simulink library "test_sequence_lib"  (R2018b)
settings: Solver=VariableStepAuto  StartTime=0.0  StopTime=10.0  RelTol=1e-3
undefined symbols (not defined in the file): C_BBU, C_DC, C_LV_BASE, C_MV_BASE, C_MV_CELL, F_NOM, ILV_MAX, ILV_MIN, IMV_MAX, IMV_MIN, INVERTER_COUNT, L_HV_BASE, L_LV_BASE, L_MV_BASE, N_CELLS_PER_STRING, N_DCDC_XFMR, N_GSU, N_MVT, plecs, r_BBU, V_LVDC_NOM, VHV_NOM, Z_HV_BASE
libraries: simulink x53, $bdroot x2
settings Model: Creator=HussamAlatrash  LastModifiedBy=ahhei
settings DataIOCC: ReturnWorkspaceOutputs=on
settings DebuggingCC: UnconnectedInputMsg=none  UnconnectedOutputMsg=none  UnconnectedLineMsg=none
settings ModelReferenceCC: EnableRefExpFcnMdlSchedulingChecks=off
settings RTWCC: Description=Generic Real-Time Target
settings ConfigComp: CovBoundaryAbsTol=1.0e-5

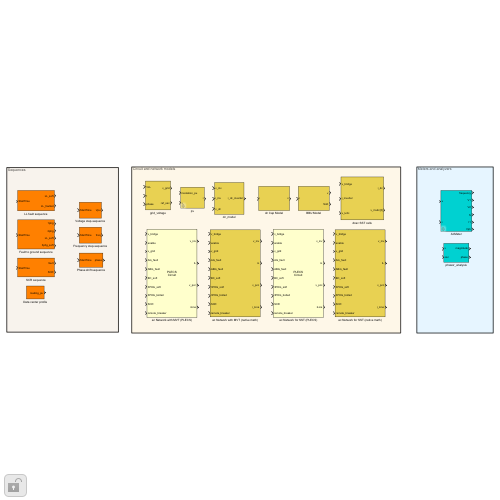
[thumbnail: Simulink's stored preview of the top-level diagram]
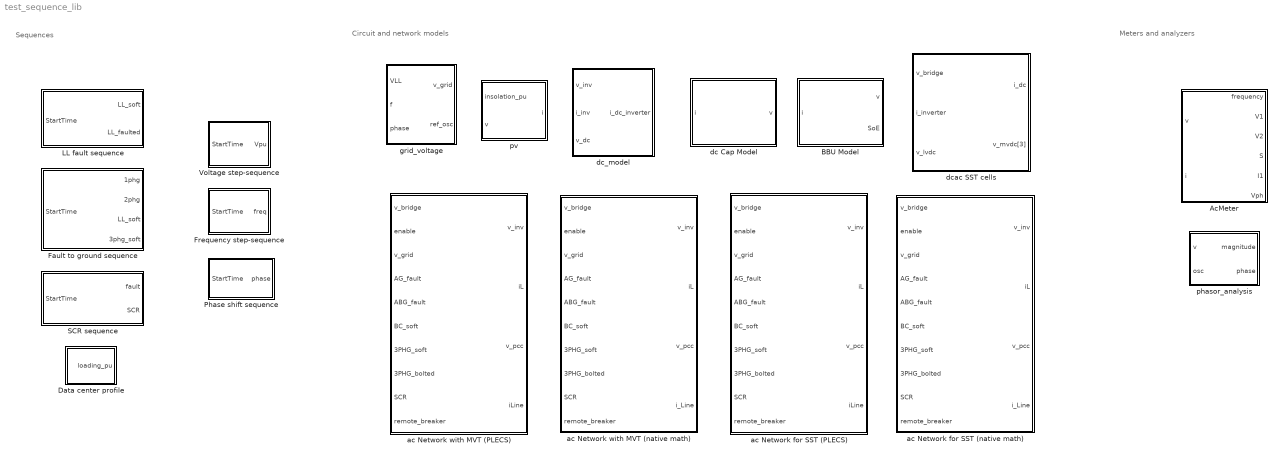
== system test_sequence_lib ==
  note: Meters and analyzers
  note: Circuit and network models
  note: Sequences
  AcMeter : Subsystem  mask{VllRated=VHV_NOM}
      mask prompts: VllRated "Rated line voltage"
  BBU Model : Subsystem
  Data center profile : Subsystem
  Fault to ground sequence : Subsystem
  Frequency step-sequence : Subsystem
  LL fault sequence : Subsystem
  Phase shift sequence : Subsystem
  SCR sequence : Subsystem
  Voltage step-sequence : Subsystem
  ac Network for SST (PLECS) : Subsystem  LoadFcn=plecs('sl', 200);  InitFcn=plecs('sl', 214);  StartFcn=plecs('sl', 208);  StopFcn=plecs('sl', 209);  mask(PlecsCircuit){PLECSData=<binary blob, 8356 chars, not shown>}
      mask prompts: PLECSData "PLECS Data (Do not delete or modify!)"
      mask init:
      | % PLACE CUSTOM INITIALIZATIONS ABOVE
      | % DO NOT REMOVE
      | plecs('sl', 215);
      | % DO NOT REMOVE
      settings: CopyFcn=plecs('sl', 203);  DeleteFcn=plecs('sl', 205);  UndoDeleteFcn=plecs('sl', 206);  PreSaveFcn=plecs('sl', 211);  PostSaveFcn=plecs('sl', 201);  NameChangeFcn=plecs('sl', 210);  DestroyFcn=plecs('sl', 207);  PreCopyFcn=plecs('sl', 216);  OpenFcn=plecs('sl', 202);  ErrorFcn=plerrorfcn
      mask Help: eval('plecs(''help'', ''qthelp:///creatingacircuit.html'')')
      mask Display: disp('PLECS\nCircuit')
  ac Network for SST (native math) : Subsystem
  ac Network with MVT (PLECS) : Subsystem  LoadFcn=plecs('sl', 200);  InitFcn=plecs('sl', 214);  StartFcn=plecs('sl', 208);  StopFcn=plecs('sl', 209);  mask(PlecsCircuit){PLECSData=<binary blob, 8620 chars, not shown>}
      mask prompts: PLECSData "PLECS Data (Do not delete or modify!)"
      mask init:
      | % PLACE CUSTOM INITIALIZATIONS ABOVE
      | % DO NOT REMOVE
      | plecs('sl', 215);
      | % DO NOT REMOVE
      settings: CopyFcn=plecs('sl', 203);  DeleteFcn=plecs('sl', 205);  UndoDeleteFcn=plecs('sl', 206);  PreSaveFcn=plecs('sl', 211);  PostSaveFcn=plecs('sl', 201);  NameChangeFcn=plecs('sl', 210);  DestroyFcn=plecs('sl', 207);  PreCopyFcn=plecs('sl', 216);  OpenFcn=plecs('sl', 202);  ErrorFcn=plerrorfcn
      mask Help: eval('plecs(''help'', ''qthelp:///creatingacircuit.html'')')
      mask Display: disp('PLECS\nCircuit')
  ac Network with MVT (native math) : Subsystem
  dc Cap Model : Subsystem
  dc_model : Subsystem
  dcac SST cells : Subsystem
  grid_voltage : Subsystem
  phasor_analysis : Subsystem
  pv : Subsystem  mask{VopenCircuit=1500, IshortCircuit=1000}
      mask prompts: VopenCircuit "Open Circuit Voltage"; IshortCircuit "Short Circuit Current"

== system test_sequence_lib/AcMeter ==
  v : Inport
  i : Inport  Port=2
  Conj : Math  Operator=conj  SaturateOnIntegerOverflow=on
  PLL_3ph : Subsystem
  Product : Product
  RMS calculator : Subsystem
  Sum of Elements : Sum  Inputs=+
  overVnom : Gain  Gain=1/VllRated
  phasor_analysis : Subsystem
  phasor_analysis1 : $bdroot/AcMeter/phasor_analysis  SystemSampleTime=-1  EmptyChoice=off  PassThrough=off  PassThroughVariantControl=(default)  EmptyChoiceVariantControl=(default)  Latency=0  AutoFrameSizeCalculation=off
  sqrt(3) : Gain  Gain=sqrt(3)
  sqrt(3)1 : Gain  Gain=sqrt(3)
  frequency : Outport
  V1 : Outport  Port=2
  V2 : Outport  Port=3
  S : Outport  Port=4
  I1 : Outport  Port=5
  Vph : Outport  Port=6
  wires:
  sqrt(3)/1 -> V1/1  "Vpve_LL"
  i/1 -> phasor_analysis1/1
  sqrt(3)1/1 -> V2/1  "Vnve_LL"
  phasor_analysis1/2 -> I1/1  "Ipve"
  phasor_analysis/3(nve) -> sqrt(3)1/1
  phasor_analysis/2(pve) -> sqrt(3)/1  "Vpve_LN"
  Product/1 -> Sum of Elements/1
  Conj/1 -> Product/2
  overVnom/1 -> PLL_3ph/1(ref)
  phasor_analysis1/1 -> Conj/1
  PLL_3ph/1(freq) -> frequency/1
  v/1 -> overVnom/1, phasor_analysis/1(in), RMS calculator/1(in[3])
  Sum of Elements/1 -> S/1  "S"
  phasor_analysis/1(perPh) -> Product/1
  PLL_3ph/2(osc[3]) -> phasor_analysis1/2, phasor_analysis/2(osc)
  RMS calculator/1(out[3]) -> Vph/1

== system test_sequence_lib/BBU Model ==
  note: this filter accounts for different caps on the bus
  i : Inport
  Constant : Constant  Value=V_LVDC_NOM
  Constant1 : Constant  Value=0.5
  Gain : Gain  Gain=4/V_LVDC_NOM
  Integrator : Integrator  InitialCondition=V_LVDC_NOM
  Saturation : Saturate  UpperLimit=1.1  LowerLimit=-0.1
  Sum : Sum  Inputs=|++
  Sum1 : Sum  Inputs=|-+
  Sum2 : Sum  Inputs=|++
  Transfer Fcn : TransferFcn  Denominator=[0.1e-3 1]
  over_BBU_capacitance : Gain  Gain=1/C_BBU
  r_BBU : Gain  Gain=r_BBU
  v : Outport
  SoE : Outport  Port=2
  wires:
  over_BBU_capacitance/1 -> Integrator/1
  Integrator/1 -> Sum/1, Sum1/2
  i/1 -> r_BBU/1, over_BBU_capacitance/1
  r_BBU/1 -> Transfer Fcn/1
  Sum/1 -> v/1
  Transfer Fcn/1 -> Sum/2
  Gain/1 -> Sum2/1
  Sum1/1 -> Gain/1
  Constant/1 -> Sum1/1
  Sum2/1 -> Saturation/1
  Constant1/1 -> Sum2/2
  Saturation/1 -> SoE/1

== system test_sequence_lib/Data center profile ==
  Compare To Constant : simulink/Logic and Bit Operations/Compare To Constant  relop=<  const=0.2  OutDataTypeStr=boolean
  Compare To Constant1 : simulink/Logic and Bit Operations/Compare To Constant  relop=<  const=0.8  OutDataTypeStr=boolean
  Compare To Constant2 : simulink/Logic and Bit Operations/Compare To Constant  relop=<  const=0.5  OutDataTypeStr=boolean
  Constant16 : Constant
  Constant17 : Constant  Value=0.1
  Constant18 : Constant  Value=0.1
  Constant19 : Constant  Value=1.5
  Floor : Rounding
  Floor1 : Rounding
  Integrator : Integrator
  Integrator1 : Integrator
  Sum : Sum  Inputs=|+-
  Sum4 : Sum  Inputs=|+-
  Switch : Switch  Criteria=u2 > Threshold
  Switch1 : Switch  Criteria=u2 > Threshold
  Switch2 : Switch  Criteria=u2 > Threshold
  cycle_frequency : Constant  Value=0.5
  pulse_frequency : Constant  Value=10
  loading_pu : Outport
  wires:
  Integrator1/1 -> Floor1/1, Sum4/1
  Floor/1 -> Sum/2
  Integrator/1 -> Sum/1, Floor/1
  Constant16/1 -> Switch/1
  Floor1/1 -> Sum4/2
  Constant17/1 -> Switch1/3  "checkpoint"
  Compare To Constant/1 -> Switch/2
  Constant18/1 -> Switch2/3
  Compare To Constant1/1 -> Switch1/2
  Sum4/1 -> Compare To Constant2/1
  Sum/1 -> Compare To Constant1/1, Compare To Constant/1
  cycle_frequency/1 -> Integrator/1
  pulse_frequency/1 -> Integrator1/1
  Switch1/1 -> Switch/3
  Compare To Constant2/1 -> Switch2/2
  Switch2/1 -> Switch1/1  "training ripple"
  Constant19/1 -> Switch2/1
  Switch/1 -> loading_pu/1

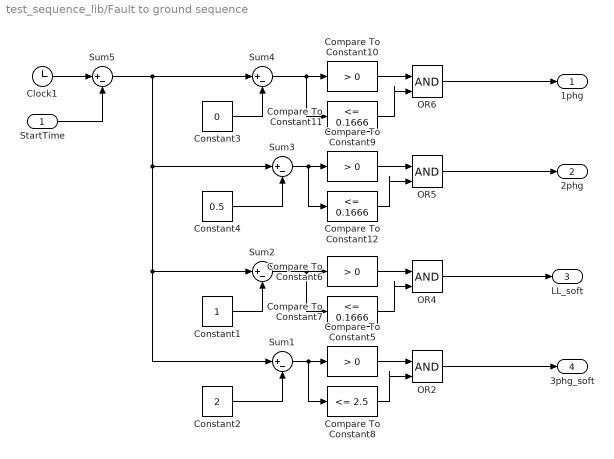
== system test_sequence_lib/Fault to ground sequence ==
  StartTime : Inport
  Clock1 : Clock
  Compare To Constant{5..6,9..10} (4 alike) : simulink/Logic and Bit Operations/Compare To Constant  relop=>  const=0  OutDataTypeStr=boolean
  Compare To Constant11 : simulink/Logic and Bit Operations/Compare To Constant  relop=<=  const=0.1666  OutDataTypeStr=boolean
  Compare To Constant12 : simulink/Logic and Bit Operations/Compare To Constant  relop=<=  const=0.1666  OutDataTypeStr=boolean
  Compare To Constant7 : simulink/Logic and Bit Operations/Compare To Constant  relop=<=  const=0.1666  OutDataTypeStr=boolean
  Compare To Constant8 : simulink/Logic and Bit Operations/Compare To Constant  relop=<=  const=2.5  OutDataTypeStr=boolean
  Constant1 : Constant
  Constant2 : Constant  Value=2
  Constant3 : Constant  Value=0
  Constant4 : Constant  Value=0.5
  OR{2,4..6} (4 alike) : Logic  IconShape=distinctive  AllPortsSameDT=off  OutDataTypeStr=boolean
  Sum{1..5} (5 alike) : Sum  Inputs=|+-
  1phg : Outport
  2phg : Outport  Port=2
  LL_soft : Outport  Port=3
  3phg_soft : Outport  Port=4
  wires:
  Compare To Constant6/1 -> OR4/1
  Compare To Constant8/1 -> OR2/2
  Compare To Constant7/1 -> OR4/2
  Sum2/1 -> Compare To Constant7/1, Compare To Constant6/1
  Sum4/1 -> Compare To Constant10/1, Compare To Constant11/1
  Constant1/1 -> Sum2/2
  Sum1/1 -> Compare To Constant8/1, Compare To Constant5/1
  Compare To Constant5/1 -> OR2/1
  Sum5/1 -> Sum4/1, Sum3/1, Sum2/1, Sum1/1
  Compare To Constant12/1 -> OR5/2
  Sum3/1 -> Compare To Constant9/1, Compare To Constant12/1
  Constant2/1 -> Sum1/2
  Compare To Constant10/1 -> OR6/1
  OR6/1 -> 1phg/1
  Compare To Constant11/1 -> OR6/2
  Compare To Constant9/1 -> OR5/1
  Constant4/1 -> Sum3/2
  Constant3/1 -> Sum4/2
  OR4/1 -> LL_soft/1
  OR5/1 -> 2phg/1
  OR2/1 -> 3phg_soft/1
  Clock1/1 -> Sum5/1
  StartTime/1 -> Sum5/2

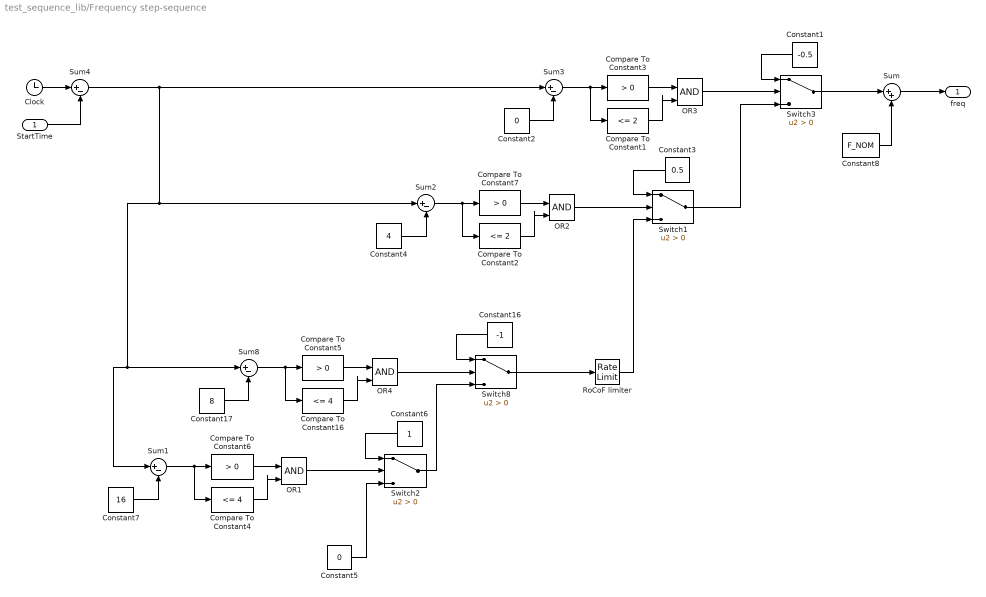
== system test_sequence_lib/Frequency step-sequence ==
  StartTime : Inport
  Clock : Clock
  Compare To Constant1 : simulink/Logic and Bit Operations/Compare To Constant  relop=<=  const=2  OutDataTypeStr=boolean
  Compare To Constant16 : simulink/Logic and Bit Operations/Compare To Constant  relop=<=  const=4  OutDataTypeStr=boolean
  Compare To Constant2 : simulink/Logic and Bit Operations/Compare To Constant  relop=<=  const=2  OutDataTypeStr=boolean
  Compare To Constant{3,5..7} (4 alike) : simulink/Logic and Bit Operations/Compare To Constant  relop=>  const=0  OutDataTypeStr=boolean
  Compare To Constant4 : simulink/Logic and Bit Operations/Compare To Constant  relop=<=  const=4  OutDataTypeStr=boolean
  Constant1 : Constant  Value=-0.5
  Constant16 : Constant  Value=-1
  Constant17 : Constant  Value=8
  Constant2 : Constant  Value=0
  Constant3 : Constant  Value=0.5
  Constant4 : Constant  Value=4
  Constant5 : Constant  Value=0
  Constant6 : Constant
  Constant7 : Constant  Value=16
  Constant8 : Constant  Value=F_NOM
  OR{1..4} (4 alike) : Logic  IconShape=distinctive  AllPortsSameDT=off  OutDataTypeStr=boolean
  RoCoF limiter : RateLimiter  SampleTimeMode=inherited
  Sum : Sum  Inputs=|++
  Sum{1..4,8} (5 alike) : Sum  Inputs=|+-
  Switch{1..3,8} (4 alike) : Switch  Criteria=u2 > Threshold
  freq : Outport
  wires:
  Switch2/1 -> Switch8/3
  Constant16/1 -> Switch8/1
  OR4/1 -> Switch8/2
  Compare To Constant5/1 -> OR4/1
  Sum8/1 -> Compare To Constant5/1, Compare To Constant16/1
  Constant17/1 -> Sum8/2
  Compare To Constant16/1 -> OR4/2
  Constant5/1 -> Switch2/3
  Constant6/1 -> Switch2/1
  OR1/1 -> Switch2/2
  Compare To Constant6/1 -> OR1/1
  Sum1/1 -> Compare To Constant6/1, Compare To Constant4/1
  Constant7/1 -> Sum1/2
  Compare To Constant4/1 -> OR1/2
  Compare To Constant2/1 -> OR2/2
  Constant4/1 -> Sum2/2
  Sum2/1 -> Compare To Constant2/1, Compare To Constant7/1
  Compare To Constant7/1 -> OR2/1
  OR2/1 -> Switch1/2
  Constant3/1 -> Switch1/1
  Switch3/1 -> Sum/1
  Compare To Constant1/1 -> OR3/2
  Constant2/1 -> Sum3/2
  Sum3/1 -> Compare To Constant1/1, Compare To Constant3/1
  Compare To Constant3/1 -> OR3/1
  OR3/1 -> Switch3/2
  Constant1/1 -> Switch3/1
  Sum4/1 -> Sum1/1, Sum8/1, Sum2/1, Sum3/1
  Switch1/1 -> Switch3/3
  Clock/1 -> Sum4/1
  StartTime/1 -> Sum4/2
  Switch8/1 -> RoCoF limiter/1
  RoCoF limiter/1 -> Switch1/3
  Sum/1 -> freq/1
  Constant8/1 -> Sum/2

== system test_sequence_lib/LL fault sequence ==
  StartTime : Inport
  Clock : Clock
  Compare To Constant1 : simulink/Logic and Bit Operations/Compare To Constant  relop=>  const=0  OutDataTypeStr=boolean
  Compare To Constant2 : simulink/Logic and Bit Operations/Compare To Constant  relop=>  const=0  OutDataTypeStr=boolean
  Compare To Constant3 : simulink/Logic and Bit Operations/Compare To Constant  relop=<=  const=0.1666  OutDataTypeStr=boolean
  Compare To Constant4 : simulink/Logic and Bit Operations/Compare To Constant  relop=<=  const=0.1666  OutDataTypeStr=boolean
  Constant11 : Constant  Value=0.5
  OR1 : Logic  IconShape=distinctive  AllPortsSameDT=off  OutDataTypeStr=boolean
  OR3 : Logic  IconShape=distinctive  AllPortsSameDT=off  OutDataTypeStr=boolean
  Sum : Sum  Inputs=|+-
  Sum8 : Sum  Inputs=|+-
  LL_soft : Outport
  LL_faulted : Outport  Port=2
  wires:
  Compare To Constant2/1 -> OR3/1
  Compare To Constant4/1 -> OR1/2
  OR1/1 -> LL_faulted/1
  Compare To Constant3/1 -> OR3/2
  OR3/1 -> LL_soft/1
  Compare To Constant1/1 -> OR1/1
  Clock/1 -> Sum/1
  StartTime/1 -> Sum/2
  Sum8/1 -> Compare To Constant1/1, Compare To Constant4/1
  Sum/1 -> Compare To Constant2/1, Compare To Constant3/1, Sum8/1
  Constant11/1 -> Sum8/2

== system test_sequence_lib/Phase shift sequence ==
  StartTime : Inport
  Clock3 : Clock
  Compare To Constant13 : simulink/Logic and Bit Operations/Compare To Constant  relop=<=  const=1  OutDataTypeStr=boolean
  Compare To Constant14 : simulink/Logic and Bit Operations/Compare To Constant  relop=>  const=0  OutDataTypeStr=boolean
  Constant5 : Constant  Value=-25*pi/180
  Constant7 : Constant  Value=0
  OR7 : Logic  IconShape=distinctive  AllPortsSameDT=off  OutDataTypeStr=boolean
  Sum5 : Sum  Inputs=|+-
  Switch3 : Switch  Criteria=u2 > Threshold
  phase : Outport
  wires:
  OR7/1 -> Switch3/2
  Sum5/1 -> Compare To Constant13/1, Compare To Constant14/1
  Constant7/1 -> Switch3/3
  Constant5/1 -> Switch3/1
  Compare To Constant14/1 -> OR7/1
  Compare To Constant13/1 -> OR7/2
  Switch3/1 -> phase/1
  Clock3/1 -> Sum5/1
  StartTime/1 -> Sum5/2

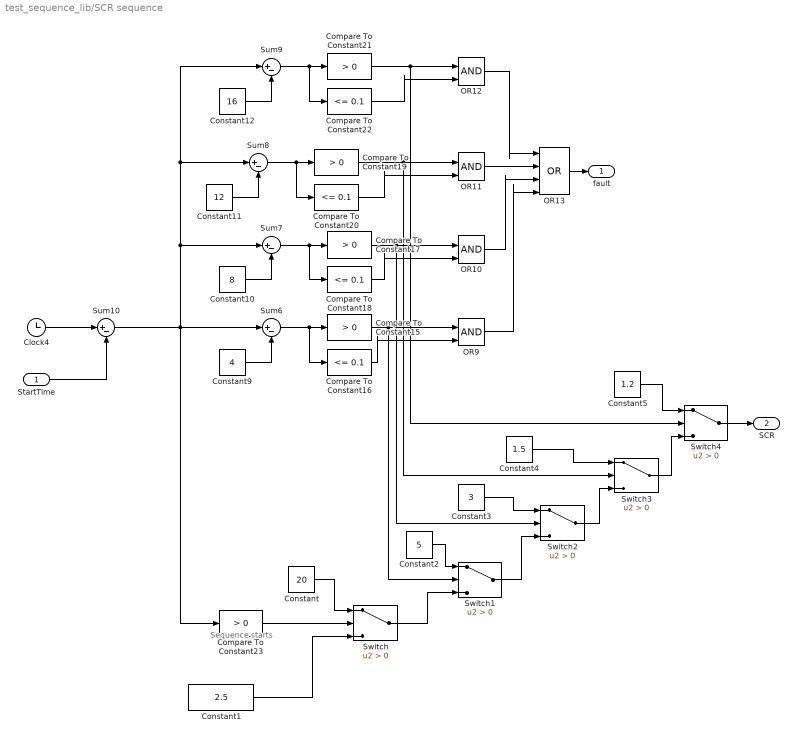
== system test_sequence_lib/SCR sequence ==
  note: Sequence starts
  StartTime : Inport
  Clock4 : Clock
  Compare To Constant{15,17,19,21,23} (5 alike) : simulink/Logic and Bit Operations/Compare To Constant  relop=>  const=0  OutDataTypeStr=boolean
  Compare To Constant{16,18,20,22} (4 alike) : simulink/Logic and Bit Operations/Compare To Constant  relop=<=  const=0.1  OutDataTypeStr=boolean
  Constant : Constant  Value=20
  Constant1 : Constant  Value=2.5
  Constant10 : Constant  Value=8
  Constant11 : Constant  Value=12
  Constant12 : Constant  Value=16
  Constant2 : Constant  Value=5
  Constant3 : Constant  Value=3
  Constant4 : Constant  Value=1.5
  Constant5 : Constant  Value=1.2
  Constant9 : Constant  Value=4
  OR{9..12} (4 alike) : Logic  IconShape=distinctive  AllPortsSameDT=off  OutDataTypeStr=boolean
  OR13 : Logic  Operator=OR  Inputs=4  IconShape=distinctive  AllPortsSameDT=off  OutDataTypeStr=boolean
  Sum{6..10} (5 alike) : Sum  Inputs=|+-
  Switch{,1..4} (5 alike) : Switch  Criteria=u2 > Threshold
  fault : Outport
  SCR : Outport  Port=2
  wires:
  OR13/1 -> fault/1
  Sum10/1 -> Sum9/1, Sum8/1, Sum7/1, Compare To Constant23/1, Sum6/1
  Constant11/1 -> Sum8/2
  Compare To Constant17/1 -> Switch2/2, OR10/1
  Sum9/1 -> Compare To Constant22/1, Compare To Constant21/1
  Clock4/1 -> Sum10/1
  Compare To Constant19/1 -> Switch3/2, OR11/1
  Sum8/1 -> Compare To Constant20/1, Compare To Constant19/1
  StartTime/1 -> Sum10/2
  Compare To Constant21/1 -> OR12/1, Switch4/2
  Compare To Constant15/1 -> Switch1/2, OR9/1
  Sum7/1 -> Compare To Constant18/1, Compare To Constant17/1
  Sum6/1 -> Compare To Constant16/1, Compare To Constant15/1
  Compare To Constant20/1 -> OR11/2
  Constant10/1 -> Sum7/2
  Compare To Constant18/1 -> OR10/2
  Constant12/1 -> Sum9/2
  Compare To Constant22/1 -> OR12/2
  Constant9/1 -> Sum6/2
  Compare To Constant16/1 -> OR9/2
  Compare To Constant23/1 -> Switch/2
  Constant/1 -> Switch/1
  Constant1/1 -> Switch/3
  Switch/1 -> Switch1/3
  OR12/1 -> OR13/1
  OR11/1 -> OR13/2
  OR10/1 -> OR13/3
  OR9/1 -> OR13/4
  Switch1/1 -> Switch2/3
  Switch2/1 -> Switch3/3
  Switch3/1 -> Switch4/3
  Constant2/1 -> Switch1/1
  Constant3/1 -> Switch2/1
  Constant4/1 -> Switch3/1
  Constant5/1 -> Switch4/1
  Switch4/1 -> SCR/1

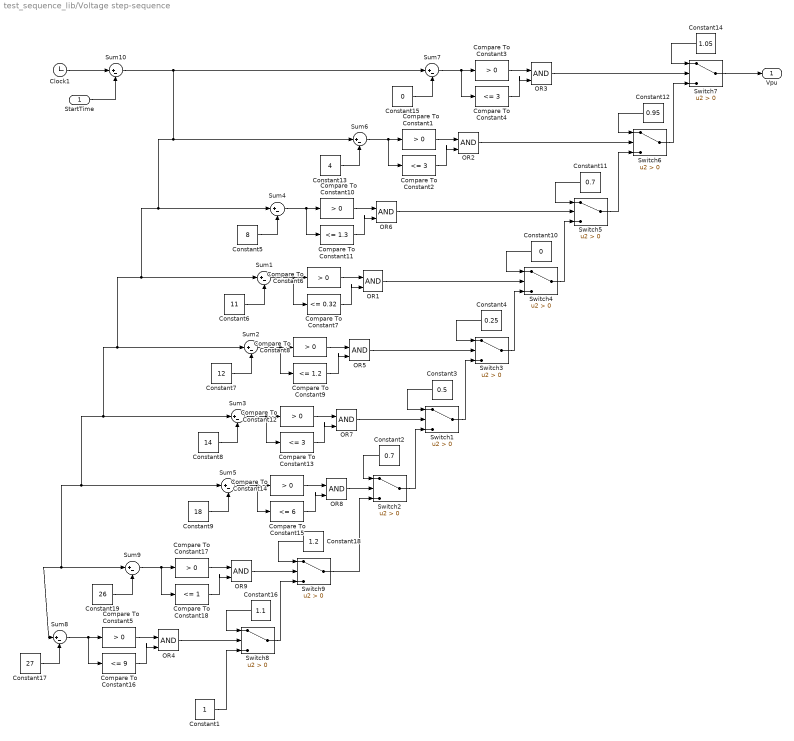
== system test_sequence_lib/Voltage step-sequence ==
  StartTime : Inport
  Clock1 : Clock
  Compare To Constant{1,3,5..6,8,10,12,14,17} (9 alike) : simulink/Logic and Bit Operations/Compare To Constant  relop=>  const=0  OutDataTypeStr=boolean
  Compare To Constant11 : simulink/Logic and Bit Operations/Compare To Constant  relop=<=  const=1.3  OutDataTypeStr=boolean
  Compare To Constant13 : simulink/Logic and Bit Operations/Compare To Constant  relop=<=  const=3  OutDataTypeStr=boolean
  Compare To Constant15 : simulink/Logic and Bit Operations/Compare To Constant  relop=<=  const=6  OutDataTypeStr=boolean
  Compare To Constant16 : simulink/Logic and Bit Operations/Compare To Constant  relop=<=  const=9  OutDataTypeStr=boolean
  Compare To Constant18 : simulink/Logic and Bit Operations/Compare To Constant  relop=<=  const=1  OutDataTypeStr=boolean
  Compare To Constant2 : simulink/Logic and Bit Operations/Compare To Constant  relop=<=  const=3  OutDataTypeStr=boolean
  Compare To Constant4 : simulink/Logic and Bit Operations/Compare To Constant  relop=<=  const=3  OutDataTypeStr=boolean
  Compare To Constant7 : simulink/Logic and Bit Operations/Compare To Constant  relop=<=  const=0.32  OutDataTypeStr=boolean
  Compare To Constant9 : simulink/Logic and Bit Operations/Compare To Constant  relop=<=  const=1.2  OutDataTypeStr=boolean
  Constant1 : Constant
  Constant10 : Constant  Value=0
  Constant11 : Constant  Value=0.7
  Constant12 : Constant  Value=0.95
  Constant13 : Constant  Value=4
  Constant14 : Constant  Value=1.05
  Constant15 : Constant  Value=0
  Constant16 : Constant  Value=1.1
  Constant17 : Constant  Value=27
  Constant18 : Constant  Value=1.2
  Constant19 : Constant  Value=26
  Constant2 : Constant  Value=0.7
  Constant3 : Constant  Value=0.5
  Constant4 : Constant  Value=0.25
  Constant5 : Constant  Value=8
  Constant6 : Constant  Value=11
  Constant7 : Constant  Value=12
  Constant8 : Constant  Value=14
  Constant9 : Constant  Value=18
  OR{1..9} (9 alike) : Logic  IconShape=distinctive  AllPortsSameDT=off  OutDataTypeStr=boolean
  Sum{1..10} (10 alike) : Sum  Inputs=|+-
  Switch{1..9} (9 alike) : Switch  Criteria=u2 > Threshold
  Vpu : Outport
  wires:
  Constant2/1 -> Switch2/1
  Switch2/1 -> Switch1/3
  Switch9/1 -> Switch2/3
  OR7/1 -> Switch1/2
  Constant3/1 -> Switch1/1
  OR8/1 -> Switch2/2
  Sum4/1 -> Compare To Constant10/1, Compare To Constant11/1
  Constant5/1 -> Sum4/2
  OR6/1 -> Switch5/2
  Compare To Constant10/1 -> OR6/1
  Compare To Constant11/1 -> OR6/2
  Compare To Constant7/1 -> OR1/2
  Compare To Constant6/1 -> OR1/1
  Constant6/1 -> Sum1/2
  Sum1/1 -> Compare To Constant7/1, Compare To Constant6/1
  Sum2/1 -> Compare To Constant8/1, Compare To Constant9/1
  Constant7/1 -> Sum2/2
  Compare To Constant8/1 -> OR5/1
  Compare To Constant9/1 -> OR5/2
  Compare To Constant13/1 -> OR7/2
  Compare To Constant12/1 -> OR7/1
  Constant8/1 -> Sum3/2
  Sum3/1 -> Compare To Constant13/1, Compare To Constant12/1
  Sum5/1 -> Compare To Constant14/1, Compare To Constant15/1
  Constant9/1 -> Sum5/2
  Compare To Constant14/1 -> OR8/1
  Compare To Constant15/1 -> OR8/2
  Constant4/1 -> Switch3/1
  OR5/1 -> Switch3/2
  OR1/1 -> Switch4/2
  Constant10/1 -> Switch4/1
  Constant11/1 -> Switch5/1
  Switch1/1 -> Switch3/3
  Switch3/1 -> Switch4/3
  Switch4/1 -> Switch5/3
  Switch5/1 -> Switch6/3
  Constant12/1 -> Switch6/1
  Compare To Constant2/1 -> OR2/2
  Compare To Constant1/1 -> OR2/1
  OR2/1 -> Switch6/2
  Constant13/1 -> Sum6/2
  Sum6/1 -> Compare To Constant2/1, Compare To Constant1/1
  Sum7/1 -> Compare To Constant3/1, Compare To Constant4/1
  Constant15/1 -> Sum7/2
  OR3/1 -> Switch7/2
  Compare To Constant3/1 -> OR3/1
  Compare To Constant4/1 -> OR3/2
  Constant14/1 -> Switch7/1
  Switch6/1 -> Switch7/3
  Switch7/1 -> Vpu/1
  Switch8/1 -> Switch9/3
  Constant18/1 -> Switch9/1
  Sum10/1 -> Sum4/1, Sum1/1, Sum2/1, Sum3/1, Sum5/1, Sum8/1, Sum9/1, Sum6/1, Sum7/1
  Compare To Constant18/1 -> OR9/2
  Compare To Constant17/1 -> OR9/1
  OR9/1 -> Switch9/2
  Constant19/1 -> Sum9/2
  Sum9/1 -> Compare To Constant18/1, Compare To Constant17/1
  Sum8/1 -> Compare To Constant5/1, Compare To Constant16/1
  Constant17/1 -> Sum8/2
  OR4/1 -> Switch8/2
  Compare To Constant5/1 -> OR4/1
  Compare To Constant16/1 -> OR4/2
  Constant16/1 -> Switch8/1
  Constant1/1 -> Switch8/3
  Clock1/1 -> Sum10/1
  StartTime/1 -> Sum10/2

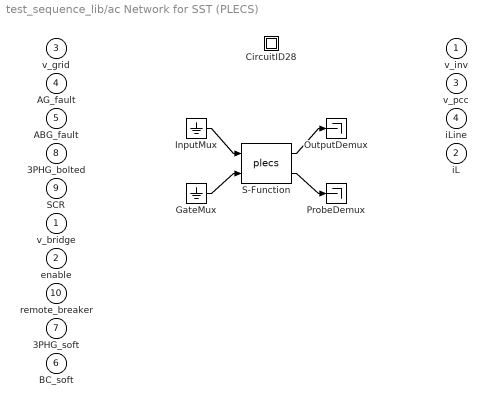
== system test_sequence_lib/ac Network for SST (PLECS) ==
  v_bridge : Inport  PortDimensions=3
  enable : Inport  Port=2  PortDimensions=1
  v_grid : Inport  Port=3  PortDimensions=3
  AG_fault : Inport  Port=4  PortDimensions=1
  ABG_fault : Inport  Port=5  PortDimensions=1
  BC_soft : Inport  Port=6  PortDimensions=1
  3PHG_soft : Inport  Port=7  PortDimensions=1
  3PHG_bolted : Inport  Port=8  PortDimensions=1
  SCR : Inport  Port=9  PortDimensions=1
  remote_breaker : Inport  Port=10  PortDimensions=1
  " CircuitID28 " : Subsystem
  " GateMux " : Ground
  " InputMux " : Ground
  " OutputDemux " : Terminator
  " ProbeDemux " : Terminator
  " S-Function " : S-Function  FunctionName=plecs  SFunctionDeploymentMode=off  EnableBusSupport=off
  v_inv : Outport  PortDimensions=3
  iL : Outport  Port=2  PortDimensions=3
  v_pcc : Outport  Port=3  PortDimensions=3
  iLine : Outport  Port=4  PortDimensions=3
  wires:
  " InputMux "/1 -> " S-Function "/1
  " GateMux "/1 -> " S-Function "/2
  " S-Function "/1 -> " OutputDemux "/1
  " S-Function "/2 -> " ProbeDemux "/1

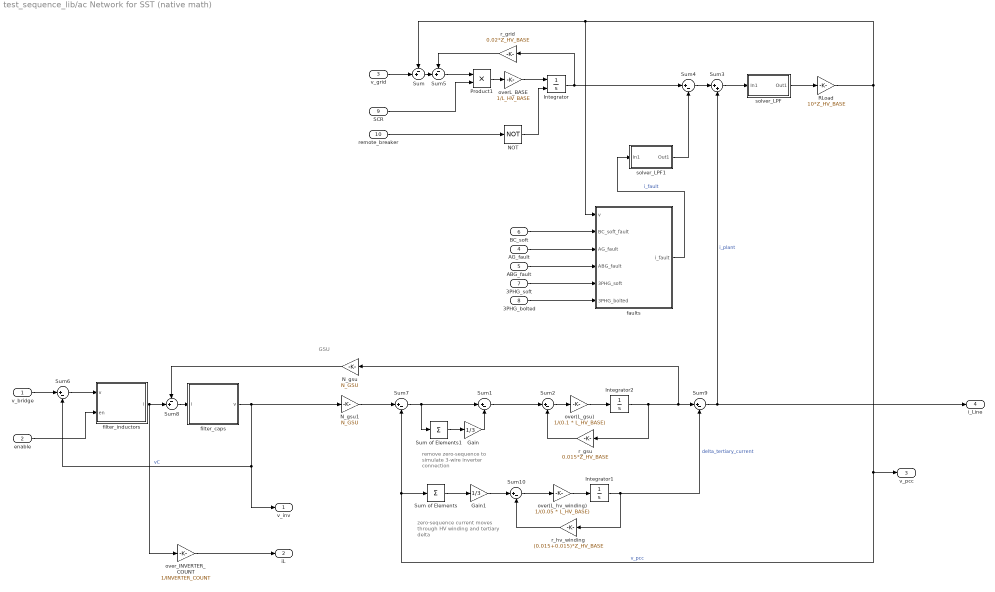
== system test_sequence_lib/ac Network for SST (native math) ==
  note: GSU
  note: remove zero-sequence to simulate 3-wire inverter connection
  note: zero-sequence current moves through HV winding and tertiary delta
  v_bridge : Inport
  enable : Inport  Port=2
  v_grid : Inport  Port=3
  AG_fault : Inport  Port=4
  ABG_fault : Inport  Port=5
  BC_soft : Inport  Port=6
  3PHG_soft : Inport  Port=7
  3PHG_bolted : Inport  Port=8
  SCR : Inport  Port=9
  remote_breaker : Inport  Port=10
  Gain : Gain  Gain=1/3
  Gain1 : Gain  Gain=1/3
  Integrator : Integrator  ExternalReset=level
  Integrator1 : Integrator
  Integrator2 : Integrator
  NOT : Logic  Operator=NOT  IconShape=distinctive  AllPortsSameDT=off  OutDataTypeStr=boolean
  N_gsu : Gain  Gain=N_GSU
  N_gsu1 : Gain  Gain=N_GSU
  Product1 : Product
  RLoad : Gain  Gain=10*Z_HV_BASE
  Sum : Sum  Inputs=-+|
  Sum of Elements : Sum  Inputs=+
  Sum of Elements1 : Sum  Inputs=+
  Sum{1..2,4,6..7,9..10} (7 alike) : Sum  Inputs=|+-
  Sum3 : Sum  Inputs=|++
  Sum5 : Sum  Inputs=-+|
  Sum8 : Sum  Inputs=-+|
  faults : Subsystem
  filter_caps : Subsystem
  filter_inductors : Subsystem
  over(L_gsu) : Gain  Gain=1/(0.1 * L_HV_BASE)
  over(L_hv_winding) : Gain  Gain=1/(0.05 * L_HV_BASE)
  overL_BASE : Gain  Gain=1/L_HV_BASE
  over_INVERTER_COUNT : Gain  Gain=1/INVERTER_COUNT
  r_grid : Gain  Gain=0.02*Z_HV_BASE
  r_gsu : Gain  Gain=0.015*Z_HV_BASE
  r_hv_winding : Gain  Gain=(0.015+0.015)*Z_HV_BASE
  solver_LPF : Subsystem
  solver_LPF1 : Subsystem
  v_inv : Outport
  iL : Outport  Port=2
  v_pcc : Outport  Port=3
  i_Line : Outport  Port=4
  wires:
  3PHG_soft/1 -> faults/5(3PHG_soft)
  Integrator2/1 -> r_gsu/1, N_gsu/1, Sum9/1
  Sum/1 -> Sum5/2
  Sum5/1 -> Product1/1
  v_grid/1 -> Sum/2
  Sum4/1 -> Sum3/1
  NOT/1 -> Integrator/2
  Sum3/1 -> solver_LPF/1(In1)
  r_grid/1 -> Sum5/1
  SCR/1 -> Product1/2
  Product1/1 -> overL_BASE/1
  v_bridge/1 -> Sum6/1
  3PHG_bolted/1 -> faults/6(3PHG_bolted)
  faults/1(i_fault) -> solver_LPF1/1(In1)  "i_fault"
  RLoad/1 -> Sum7/2, Sum of Elements/1, v_pcc/1, Sum/1, faults/1(v)  "v_pcc"
  solver_LPF1/1(Out1) -> Sum4/2
  Integrator/1 -> r_grid/1, Sum4/1
  overL_BASE/1 -> Integrator/1
  remote_breaker/1 -> NOT/1
  solver_LPF/1(Out1) -> RLoad/1
  over(L_gsu)/1 -> Integrator2/1
  Sum7/1 -> Sum of Elements1/1, Sum1/1
  Sum2/1 -> over(L_gsu)/1
  Sum of Elements1/1 -> Gain/1
  Gain/1 -> Sum1/2
  Sum1/1 -> Sum2/1
  r_gsu/1 -> Sum2/2
  Sum6/1 -> filter_inductors/1(v)
  enable/1 -> filter_inductors/2(en)
  filter_inductors/1(i) -> Sum8/2, over_INVERTER_COUNT/1
  Sum8/1 -> filter_caps/1(i)
  filter_caps/1(v) -> v_inv/1, Sum6/2, N_gsu1/1  "vC"
  over_INVERTER_COUNT/1 -> iL/1
  N_gsu1/1 -> Sum7/1
  N_gsu/1 -> Sum8/1
  Sum9/1 -> Sum3/2, i_Line/1  "i_plant"
  over(L_hv_winding)/1 -> Integrator1/1
  Integrator1/1 -> Sum9/2, r_hv_winding/1  "delta_tertiary_current"
  r_hv_winding/1 -> Sum10/2
  Sum10/1 -> over(L_hv_winding)/1
  Sum of Elements/1 -> Gain1/1
  Gain1/1 -> Sum10/1
  BC_soft/1 -> faults/2(BC_soft_fault)
  ABG_fault/1 -> faults/4(ABG_fault)
  AG_fault/1 -> faults/3(AG_fault)

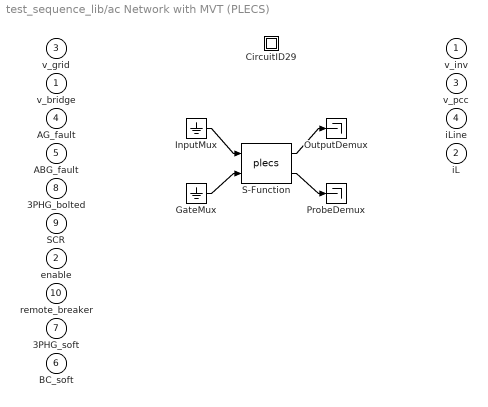
== system test_sequence_lib/ac Network with MVT (PLECS) ==
  v_bridge : Inport  PortDimensions=3
  enable : Inport  Port=2  PortDimensions=1
  v_grid : Inport  Port=3  PortDimensions=3
  AG_fault : Inport  Port=4  PortDimensions=1
  ABG_fault : Inport  Port=5  PortDimensions=1
  BC_soft : Inport  Port=6  PortDimensions=1
  3PHG_soft : Inport  Port=7  PortDimensions=1
  3PHG_bolted : Inport  Port=8  PortDimensions=1
  SCR : Inport  Port=9  PortDimensions=1
  remote_breaker : Inport  Port=10  PortDimensions=1
  " CircuitID29 " : Subsystem
  " GateMux " : Ground
  " InputMux " : Ground
  " OutputDemux " : Terminator
  " ProbeDemux " : Terminator
  " S-Function " : S-Function  FunctionName=plecs  SFunctionDeploymentMode=off  EnableBusSupport=off
  v_inv : Outport  PortDimensions=3
  iL : Outport  Port=2  PortDimensions=3
  v_pcc : Outport  Port=3  PortDimensions=3
  iLine : Outport  Port=4  PortDimensions=3
  wires:
  " InputMux "/1 -> " S-Function "/1
  " GateMux "/1 -> " S-Function "/2
  " S-Function "/1 -> " OutputDemux "/1
  " S-Function "/2 -> " ProbeDemux "/1

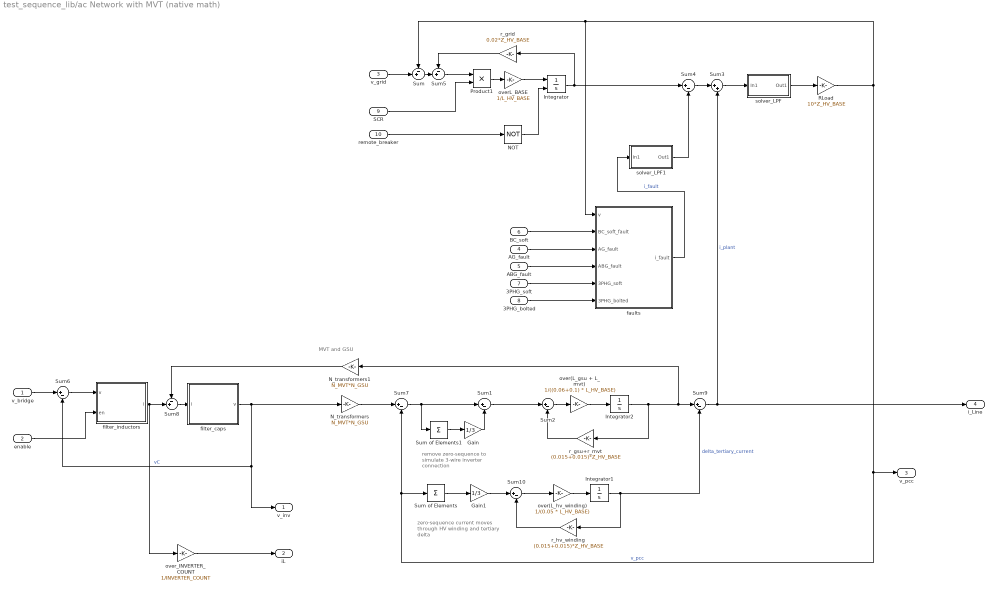
== system test_sequence_lib/ac Network with MVT (native math) ==
  note: MVT and GSU
  note: remove zero-sequence to simulate 3-wire inverter connection
  note: zero-sequence current moves through HV winding and tertiary delta
  v_bridge : Inport
  enable : Inport  Port=2
  v_grid : Inport  Port=3
  AG_fault : Inport  Port=4
  ABG_fault : Inport  Port=5
  BC_soft : Inport  Port=6
  3PHG_soft : Inport  Port=7
  3PHG_bolted : Inport  Port=8
  SCR : Inport  Port=9
  remote_breaker : Inport  Port=10
  Gain : Gain  Gain=1/3
  Gain1 : Gain  Gain=1/3
  Integrator : Integrator  ExternalReset=level
  Integrator1 : Integrator
  Integrator2 : Integrator
  NOT : Logic  Operator=NOT  IconShape=distinctive  AllPortsSameDT=off  OutDataTypeStr=boolean
  N_transformers : Gain  Gain=N_MVT*N_GSU
  N_transformers1 : Gain  Gain=N_MVT*N_GSU
  Product1 : Product
  RLoad : Gain  Gain=10*Z_HV_BASE
  Sum : Sum  Inputs=-+|
  Sum of Elements : Sum  Inputs=+
  Sum of Elements1 : Sum  Inputs=+
  Sum{1..2,4,6..7,9..10} (7 alike) : Sum  Inputs=|+-
  Sum3 : Sum  Inputs=|++
  Sum5 : Sum  Inputs=-+|
  Sum8 : Sum  Inputs=-+|
  faults : Subsystem
  filter_caps : Subsystem
  filter_inductors : Subsystem
  over(L_gsu + L_mvt) : Gain  Gain=1/((0.06+0.1) * L_HV_BASE)
  over(L_hv_winding) : Gain  Gain=1/(0.05 * L_HV_BASE)
  overL_BASE : Gain  Gain=1/L_HV_BASE
  over_INVERTER_COUNT : Gain  Gain=1/INVERTER_COUNT
  r_grid : Gain  Gain=0.02*Z_HV_BASE
  r_gsu+r_mvt : Gain  Gain=(0.015+0.015)*Z_HV_BASE
  r_hv_winding : Gain  Gain=(0.015+0.015)*Z_HV_BASE
  solver_LPF : Subsystem
  solver_LPF1 : Subsystem
  v_inv : Outport
  iL : Outport  Port=2
  v_pcc : Outport  Port=3
  i_Line : Outport  Port=4
  wires:
  3PHG_soft/1 -> faults/5(3PHG_soft)
  Integrator2/1 -> r_gsu+r_mvt/1, N_transformers1/1, Sum9/1
  Sum/1 -> Sum5/2
  Sum5/1 -> Product1/1
  v_grid/1 -> Sum/2
  Sum4/1 -> Sum3/1
  NOT/1 -> Integrator/2
  Sum3/1 -> solver_LPF/1(In1)
  r_grid/1 -> Sum5/1
  SCR/1 -> Product1/2
  Product1/1 -> overL_BASE/1
  v_bridge/1 -> Sum6/1
  3PHG_bolted/1 -> faults/6(3PHG_bolted)
  faults/1(i_fault) -> solver_LPF1/1(In1)  "i_fault"
  RLoad/1 -> Sum7/2, Sum of Elements/1, v_pcc/1, Sum/1, faults/1(v)  "v_pcc"
  solver_LPF1/1(Out1) -> Sum4/2
  Integrator/1 -> r_grid/1, Sum4/1
  overL_BASE/1 -> Integrator/1
  remote_breaker/1 -> NOT/1
  solver_LPF/1(Out1) -> RLoad/1
  over(L_gsu + L_mvt)/1 -> Integrator2/1
  Sum7/1 -> Sum of Elements1/1, Sum1/1
  Sum2/1 -> over(L_gsu + L_mvt)/1
  Sum of Elements1/1 -> Gain/1
  Gain/1 -> Sum1/2
  Sum1/1 -> Sum2/1
  r_gsu+r_mvt/1 -> Sum2/2
  Sum6/1 -> filter_inductors/1(v)
  enable/1 -> filter_inductors/2(en)
  filter_inductors/1(i) -> Sum8/2, over_INVERTER_COUNT/1
  Sum8/1 -> filter_caps/1(i)
  filter_caps/1(v) -> v_inv/1, Sum6/2, N_transformers/1  "vC"
  over_INVERTER_COUNT/1 -> iL/1
  N_transformers/1 -> Sum7/1
  N_transformers1/1 -> Sum8/1
  Sum9/1 -> Sum3/2, i_Line/1  "i_plant"
  over(L_hv_winding)/1 -> Integrator1/1
  Integrator1/1 -> Sum9/2, r_hv_winding/1  "delta_tertiary_current"
  r_hv_winding/1 -> Sum10/2
  Sum10/1 -> over(L_hv_winding)/1
  Sum of Elements/1 -> Gain1/1
  Gain1/1 -> Sum10/1
  BC_soft/1 -> faults/2(BC_soft_fault)
  ABG_fault/1 -> faults/4(ABG_fault)
  AG_fault/1 -> faults/3(AG_fault)

== system test_sequence_lib/dc Cap Model ==
  i : Inport
  Integrator : Integrator  InitialCondition=V_LVDC_NOM
  over_capacitance : Gain  Gain=1/C_DC
  v : Outport
  wires:
  over_capacitance/1 -> Integrator/1
  i/1 -> over_capacitance/1
  Integrator/1 -> v/1

== system test_sequence_lib/dc_model ==
  v_inv : Inport
  i_inv : Inport  Port=2
  v_dc : Inport  Port=3
  Product : Product
  Product1 : Product  Inputs=*/
  Saturation : Saturate  UpperLimit=inf  LowerLimit=10
  Sum of Elements : Sum  Inputs=+
  i_dc_inverter : Outport
  wires:
  v_dc/1 -> Saturation/1
  Sum of Elements/1 -> Product1/1  "P_ac"
  i_inv/1 -> Product/2
  Product/1 -> Sum of Elements/1
  Product1/1 -> i_dc_inverter/1  "i_dc_inverter"
  v_inv/1 -> Product/1
  Saturation/1 -> Product1/2

== system test_sequence_lib/dcac SST cells ==
  note: The three aggregate dc-bus voltages for the three phases do not naturally balance and need this algorithm to do so
  v_bridge : Inport
  i_inverter : Inport  Port=2
  v_lvdc : Inport  Port=3
  Gain1 : Gain  Gain=1/3
  N_cells : Gain  Gain=N_CELLS_PER_STRING
  N_cells1 : Gain  Gain=N_CELLS_PER_STRING
  SST Cell Model : Subsystem
  Sum of Elements : Sum  Inputs=+
  Sum of Elements1 : Sum  Inputs=+
  Sum4 : Sum  Inputs=-+|
  dcdcController : Subsystem
  kRebalance : Gain  Gain=5
  over_N_cells : Gain  Gain=1/N_CELLS_PER_STRING
  i_dc : Outport
  v_mvdc[3] : Outport  Port=2
  wires:
  kRebalance/1 -> dcdcController/3(P_dcdc_ffwd)  "p_string_rebalance"
  N_cells1/1 -> Sum of Elements/1
  N_cells/1 -> v_mvdc[3]/1, Sum4/1, Sum of Elements1/1  "v_mvdc_bus"
  Sum4/1 -> kRebalance/1
  SST Cell Model/2(i_LV) -> N_cells1/1
  Sum of Elements1/1 -> Gain1/1
  dcdcController/1(i_MV_ref) -> SST Cell Model/2(i_MV)
  Gain1/1 -> Sum4/2
  SST Cell Model/1(v_MV_cell) -> N_cells/1, dcdcController/2(v_MV_cell)  "v_mvdc_cell"
  over_N_cells/1 -> SST Cell Model/3(v_ac)
  v_lvdc/1 -> SST Cell Model/1(v_LV), dcdcController/1(v_LV)
  v_bridge/1 -> over_N_cells/1
  Sum of Elements/1 -> i_dc/1  "I_dc_sst"
  i_inverter/1 -> SST Cell Model/4(i_ac)

== system test_sequence_lib/grid_voltage ==
  VLL : Inport
  f : Inport  Port=2
  phase : Inport  Port=3
  Complex to Real-Imag : ComplexToRealImag
  Gain : Gain  Gain=sqrt(2)
  Gain1 : Gain  Gain=1/sqrt(3)
  Product : Product
  oscillator_3ph : Subsystem
  v_grid : Outport
  ref_osc : Outport  Port=2
  wires:
  Complex to Real-Imag/1 -> Gain/1
  oscillator_3ph/1(osc[3]) -> ref_osc/1, Complex to Real-Imag/1
  f/1 -> oscillator_3ph/1(f)
  Gain/1 -> Product/1
  Product/1 -> Gain1/1
  Gain1/1 -> v_grid/1
  VLL/1 -> Product/2
  phase/1 -> oscillator_3ph/2(phase)

== system test_sequence_lib/phasor_analysis ==
  v : Inport
  osc : Inport  Port=2
  Complex to Magnitude-Angle : ComplexToMagnitudeAngle
  Complex to Real-Imag : ComplexToRealImag
  Conj : Math  Operator=conj  SaturateOnIntegerOverflow=on
  Gain : Gain  Gain=sqrt(2)
  Gain1 : Gain  Gain=1/3
  Gain2 : Gain  Gain=sqrt(3)
  Product3 : Product
  Real-Imag to Complex : RealImagToComplex
  Sum of Elements1 : Sum  Inputs=+
  Transfer Fcn : TransferFcn  Denominator=[0.01 1]
  Transfer Fcn1 : TransferFcn  Denominator=[0.01 1]
  magnitude : Outport
  phase : Outport  Port=2
  wires:
  Transfer Fcn1/1 -> Real-Imag to Complex/2
  Sum of Elements1/1 -> Gain1/1
  Transfer Fcn/1 -> Real-Imag to Complex/1
  Product3/1 -> Sum of Elements1/1
  Complex to Real-Imag/2 -> Transfer Fcn1/1
  v/1 -> Product3/1
  Complex to Real-Imag/1 -> Transfer Fcn/1
  osc/1 -> Conj/1
  Conj/1 -> Gain/1
  Real-Imag to Complex/1 -> Gain2/1
  Gain/1 -> Product3/2
  Gain1/1 -> Complex to Real-Imag/1
  Gain2/1 -> Complex to Magnitude-Angle/1
  Complex to Magnitude-Angle/1 -> magnitude/1
  Complex to Magnitude-Angle/2 -> phase/1

== system test_sequence_lib/pv ==
  insolation_pu : Inport
  v : Inport  Port=2
  Exp : Math  SaturateOnIntegerOverflow=on
  Inom : Gain  Gain=IshortCircuit
  Sum3 : Sum  Inputs=|+-
  Sum4 : Sum  Inputs=|+-
  Voc_normalized : Constant
  diode : Saturate  Commented=through  UpperLimit=inf  LowerLimit=0
  overVnom : Gain  Gain=1/VopenCircuit
  overVt : Gain  Gain=1/0.1
  i : Outport
  wires:
  diode/1 -> Inom/1
  Inom/1 -> i/1
  overVnom/1 -> Sum4/1
  insolation_pu/1 -> Sum3/1
  Sum3/1 -> diode/1
  Exp/1 -> Sum3/2
  overVt/1 -> Exp/1
  Sum4/1 -> overVt/1
  v/1 -> overVnom/1
  Voc_normalized/1 -> Sum4/2

== system test_sequence_lib/AcMeter/PLL_3ph ==
  ref : Inport
  Complex to Real-Imag : ComplexToRealImag
  Conj : Math  Operator=conj  SaturateOnIntegerOverflow=on
  Constant : Constant  Value=120
  Gain1 : Gain  Gain=1.5
  Gain2 : Gain  Gain=4.5
  Gain3 : Gain  Gain=10e-3
  Integrator : Integrator  LimitOutput=on  UpperSaturationLimit=5  LowerSaturationLimit=-5
  Product : Product
  SOGI : Subsystem  AncestorBlock=controls_module_lib/dcVoltageRegulator_A/SOGI
  Saturation : Saturate  UpperLimit=5  LowerLimit=-5
  Sum : Sum  Inputs=+++
  Sum of Elements : Sum  Inputs=+
  Sum1 : Sum  Inputs=|+-
  Transfer Fcn : TransferFcn  Denominator=[0.02 1]
  f_nom : Constant  Value=60
  oscillator_3ph : Subsystem
  freq : Outport
  osc[3] : Outport  Port=2
  wires:
  Constant/1 -> SOGI/2(fnom)
  Transfer Fcn/1 -> SOGI/1(in)  "phase_error"
  f_nom/1 -> Sum/1
  Gain3/1 -> Sum1/2
  Sum of Elements/1 -> Transfer Fcn/1
  SOGI/1(notch) -> Gain1/1, Gain2/1  "phase_error"
  Saturation/1 -> Sum/2
  Product/1 -> Sum of Elements/1
  Sum/1 -> freq/1, oscillator_3ph/1(f)  "freq"
  oscillator_3ph/1(osc[3]) -> Conj/1, osc[3]/1
  Gain2/1 -> Sum1/1
  Complex to Real-Imag/2 -> Product/2
  Sum1/1 -> Integrator/1
  Integrator/1 -> Gain3/1, Sum/3
  ref/1 -> Product/1
  Conj/1 -> Complex to Real-Imag/1
  Gain1/1 -> Saturation/1

== system test_sequence_lib/AcMeter/RMS calculator ==
  in[3] : Inport
  Gain : Gain  Gain=20
  Integrator : Integrator
  Square : Math  Operator=square  SaturateOnIntegerOverflow=on
  Square Root : Sqrt  SaturateOnIntegerOverflow=on
  Sum : Sum  Inputs=|+-
  out[3] : Outport
  wires:
  Integrator/1 -> Sum/2, Square Root/1
  Sum/1 -> Gain/1
  Square Root/1 -> out[3]/1  "Vph_rms"
  Gain/1 -> Integrator/1
  Square/1 -> Sum/1
  in[3]/1 -> Square/1

== system test_sequence_lib/AcMeter/phasor_analysis ==
  in : Inport
  osc : Inport  Port=2
  Conj : Math  Operator=conj  SaturateOnIntegerOverflow=on
  Conj1 : Math  Operator=conj  SaturateOnIntegerOverflow=on
  Demux : Demux  Outputs=3
  Gain1 : Gain  Gain=1/3
  Gain3 : Gain  Gain=1/3
  Mux : Mux  Inputs=3
  Product1 : Product
  Product3 : Product
  Sum of Elements1 : Sum  Inputs=+
  Sum of Elements2 : Sum  Inputs=+
  complex_LPF1 : Subsystem  mask{wLPF=50}
      mask prompts: wLPF "Bandwidth (rad/sec)"
  complex_LPF2 : $bdroot/AcMeter/phasor_analysis/complex_LPF1  wLPF=50
  sqrt(2) : Gain  Gain=sqrt(2)
  sqrt(2)1 : Gain  Gain=sqrt(2)
  perPh : Outport
  pve : Outport  Port=2
  nve : Outport  Port=3
  wires:
  Gain3/1 -> nve/1
  Sum of Elements2/1 -> Gain3/1
  sqrt(2)1/1 -> Product1/2
  Conj1/1 -> sqrt(2)1/1
  Mux/1 -> Conj1/1
  Demux/3 -> Mux/2
  Demux/2 -> Mux/3
  Demux/1 -> Mux/1
  Gain1/1 -> pve/1
  sqrt(2)/1 -> Product3/2
  Conj/1 -> sqrt(2)/1
  osc/1 -> Conj/1, Demux/1
  in/1 -> Product1/1, Product3/1
  Sum of Elements1/1 -> Gain1/1
  Product3/1 -> complex_LPF1/1(In1)
  complex_LPF1/1(1) -> Sum of Elements1/1, perPh/1
  Product1/1 -> complex_LPF2/1
  complex_LPF2/1 -> Sum of Elements2/1

== system test_sequence_lib/ac Network for SST (PLECS)/ CircuitID28  ==

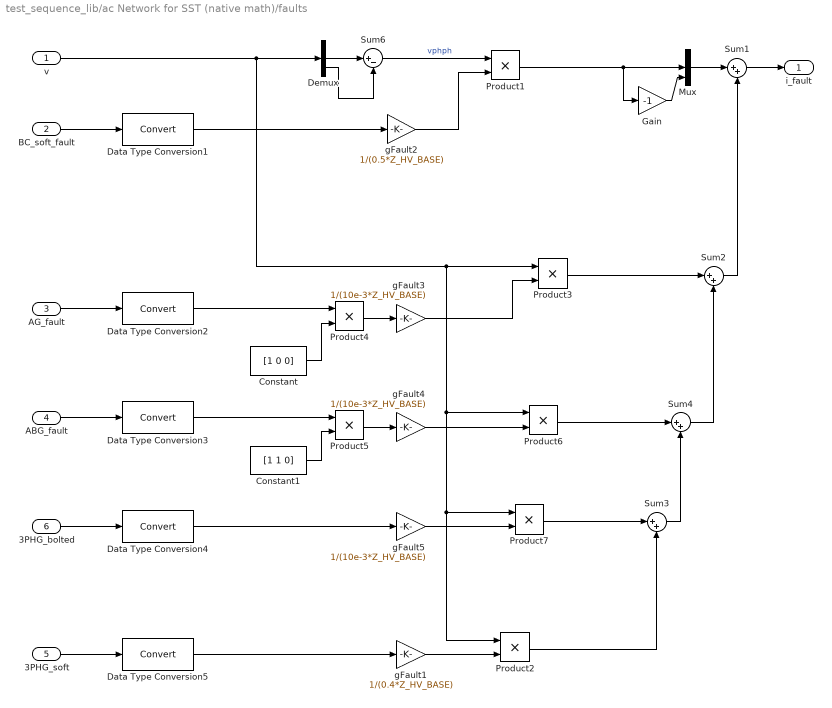
== system test_sequence_lib/ac Network for SST (native math)/faults ==
  v : Inport
  BC_soft_fault : Inport  Port=2
  AG_fault : Inport  Port=3
  ABG_fault : Inport  Port=4
  3PHG_soft : Inport  Port=5
  3PHG_bolted : Inport  Port=6
  Constant : Constant  Value=[1 0 0]
  Constant1 : Constant  Value=[1 1 0]
  Data Type Conversion{1..5} (5 alike) : DataTypeConversion
  Demux : Demux  Outputs=3
  Gain : Gain  Gain=-1
  Mux : Mux  Inputs=3
  Product{1..7} (7 alike) : Product
  Sum{1..4} (4 alike) : Sum  Inputs=|++
  Sum6 : Sum  Inputs=|+-
  gFault1 : Gain  Gain=1/(0.4*Z_HV_BASE)
  gFault2 : Gain  Gain=1/(0.5*Z_HV_BASE)
  gFault3 : Gain  Gain=1/(10e-3*Z_HV_BASE)
  gFault4 : Gain  Gain=1/(10e-3*Z_HV_BASE)
  gFault5 : Gain  Gain=1/(10e-3*Z_HV_BASE)
  i_fault : Outport
  wires:
  Data Type Conversion5/1 -> gFault1/1
  Data Type Conversion4/1 -> gFault5/1
  Data Type Conversion3/1 -> Product5/1
  Data Type Conversion2/1 -> Product4/1
  Data Type Conversion1/1 -> gFault2/1
  Sum3/1 -> Sum4/2
  Product7/1 -> Sum3/1
  Sum4/1 -> Sum2/2
  Product6/1 -> Sum4/1
  Sum2/1 -> Sum1/2
  3PHG_soft/1 -> Data Type Conversion5/1
  3PHG_bolted/1 -> Data Type Conversion4/1
  ABG_fault/1 -> Data Type Conversion3/1
  AG_fault/1 -> Data Type Conversion2/1
  BC_soft_fault/1 -> Data Type Conversion1/1
  gFault5/1 -> Product7/2
  gFault4/1 -> Product6/2
  Product3/1 -> Sum2/1
  Product5/1 -> gFault4/1
  Constant1/1 -> Product5/2
  Constant/1 -> Product4/2
  Product4/1 -> gFault3/1
  Mux/1 -> Sum1/1
  gFault3/1 -> Product3/2
  gFault2/1 -> Product1/2
  Sum6/1 -> Product1/1  "vphph"
  Gain/1 -> Mux/3
  Demux/2 -> Sum6/1
  Demux/3 -> Sum6/2
  v/1 -> Product2/1, Product7/1, Product6/1, Product3/1, Demux/1
  Product1/1 -> Mux/2, Gain/1
  Sum1/1 -> i_fault/1
  gFault1/1 -> Product2/2
  Product2/1 -> Sum3/2

== system test_sequence_lib/ac Network for SST (native math)/filter_caps ==
  i : Inport
  Gain1 : Gain  Gain=1/(0.03*C_MV_BASE)
  Integrator1 : Integrator
  v : Outport
  wires:
  i/1 -> Gain1/1
  Integrator1/1 -> v/1
  Gain1/1 -> Integrator1/1

== system test_sequence_lib/ac Network for SST (native math)/filter_inductors ==
  v : Inport
  en : Inport  Port=2
  Gain1 : Gain  Gain=1/(0.02*L_MV_BASE)
  Integrator1 : Integrator  ExternalReset=level
  NOT : Logic  Operator=NOT  IconShape=distinctive  AllPortsSameDT=off  OutDataTypeStr=boolean
  i : Outport
  wires:
  en/1 -> NOT/1
  Gain1/1 -> Integrator1/1
  Integrator1/1 -> i/1
  v/1 -> Gain1/1
  NOT/1 -> Integrator1/2

== system test_sequence_lib/ac Network for SST (native math)/solver_LPF ==
  In1 : Inport
  Gain : Gain  Gain=1/50e-6
  Integrator1 : Integrator
  Sum1 : Sum  Inputs=|+-
  Out1 : Outport
  wires:
  In1/1 -> Sum1/1
  Integrator1/1 -> Sum1/2, Out1/1
  Sum1/1 -> Gain/1
  Gain/1 -> Integrator1/1

== system test_sequence_lib/ac Network for SST (native math)/solver_LPF1 ==
  In1 : Inport
  Gain : Gain  Gain=1/1e-3
  Integrator1 : Integrator
  Sum1 : Sum  Inputs=|+-
  Out1 : Outport
  wires:
  Gain/1 -> Integrator1/1
  Sum1/1 -> Gain/1
  Integrator1/1 -> Out1/1, Sum1/2
  In1/1 -> Sum1/1

== system test_sequence_lib/ac Network with MVT (PLECS)/ CircuitID29  ==

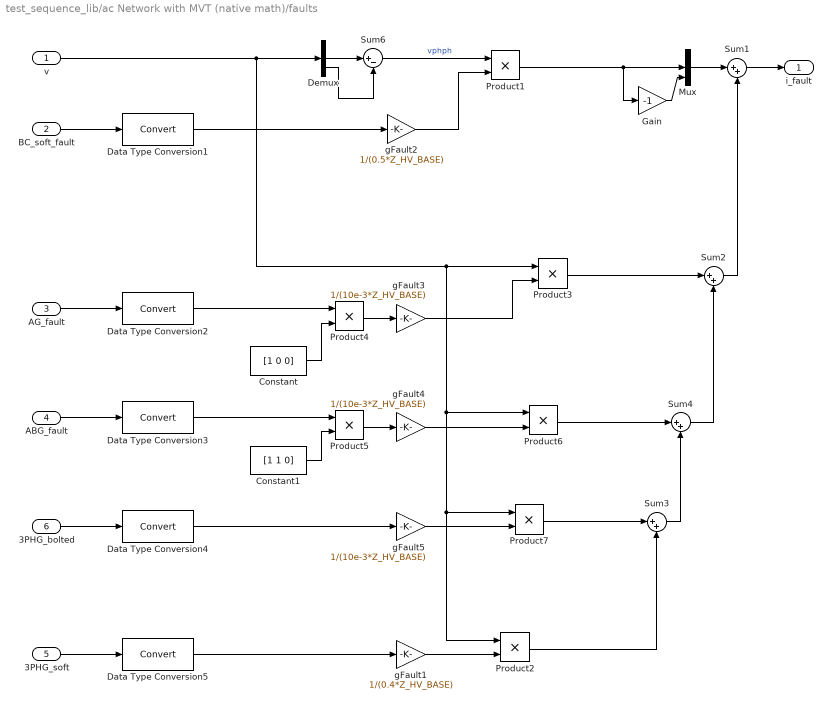
== system test_sequence_lib/ac Network with MVT (native math)/faults ==
  v : Inport
  BC_soft_fault : Inport  Port=2
  AG_fault : Inport  Port=3
  ABG_fault : Inport  Port=4
  3PHG_soft : Inport  Port=5
  3PHG_bolted : Inport  Port=6
  Constant : Constant  Value=[1 0 0]
  Constant1 : Constant  Value=[1 1 0]
  Data Type Conversion{1..5} (5 alike) : DataTypeConversion
  Demux : Demux  Outputs=3
  Gain : Gain  Gain=-1
  Mux : Mux  Inputs=3
  Product{1..7} (7 alike) : Product
  Sum{1..4} (4 alike) : Sum  Inputs=|++
  Sum6 : Sum  Inputs=|+-
  gFault1 : Gain  Gain=1/(0.4*Z_HV_BASE)
  gFault2 : Gain  Gain=1/(0.5*Z_HV_BASE)
  gFault3 : Gain  Gain=1/(10e-3*Z_HV_BASE)
  gFault4 : Gain  Gain=1/(10e-3*Z_HV_BASE)
  gFault5 : Gain  Gain=1/(10e-3*Z_HV_BASE)
  i_fault : Outport
  wires:
  Data Type Conversion5/1 -> gFault1/1
  Data Type Conversion4/1 -> gFault5/1
  Data Type Conversion3/1 -> Product5/1
  Data Type Conversion2/1 -> Product4/1
  Data Type Conversion1/1 -> gFault2/1
  Sum3/1 -> Sum4/2
  Product7/1 -> Sum3/1
  Sum4/1 -> Sum2/2
  Product6/1 -> Sum4/1
  Sum2/1 -> Sum1/2
  3PHG_soft/1 -> Data Type Conversion5/1
  3PHG_bolted/1 -> Data Type Conversion4/1
  ABG_fault/1 -> Data Type Conversion3/1
  AG_fault/1 -> Data Type Conversion2/1
  BC_soft_fault/1 -> Data Type Conversion1/1
  gFault5/1 -> Product7/2
  gFault4/1 -> Product6/2
  Product3/1 -> Sum2/1
  Product5/1 -> gFault4/1
  Constant1/1 -> Product5/2
  Constant/1 -> Product4/2
  Product4/1 -> gFault3/1
  Mux/1 -> Sum1/1
  gFault3/1 -> Product3/2
  gFault2/1 -> Product1/2
  Sum6/1 -> Product1/1  "vphph"
  Gain/1 -> Mux/3
  Demux/2 -> Sum6/1
  Demux/3 -> Sum6/2
  v/1 -> Product2/1, Product7/1, Product6/1, Product3/1, Demux/1
  Product1/1 -> Mux/2, Gain/1
  Sum1/1 -> i_fault/1
  gFault1/1 -> Product2/2
  Product2/1 -> Sum3/2

== system test_sequence_lib/ac Network with MVT (native math)/filter_caps ==
  i : Inport
  Gain1 : Gain  Gain=1/(0.03*C_LV_BASE)
  Integrator1 : Integrator
  v : Outport
  wires:
  i/1 -> Gain1/1
  Integrator1/1 -> v/1
  Gain1/1 -> Integrator1/1

== system test_sequence_lib/ac Network with MVT (native math)/filter_inductors ==
  v : Inport
  en : Inport  Port=2
  Gain1 : Gain  Gain=1/(0.02*L_LV_BASE)
  Integrator1 : Integrator  ExternalReset=level
  NOT : Logic  Operator=NOT  IconShape=distinctive  AllPortsSameDT=off  OutDataTypeStr=boolean
  i : Outport
  wires:
  en/1 -> NOT/1
  Gain1/1 -> Integrator1/1
  Integrator1/1 -> i/1
  v/1 -> Gain1/1
  NOT/1 -> Integrator1/2

== system test_sequence_lib/ac Network with MVT (native math)/solver_LPF ==
  In1 : Inport
  Gain : Gain  Gain=1/50e-6
  Integrator1 : Integrator
  Sum1 : Sum  Inputs=|+-
  Out1 : Outport
  wires:
  In1/1 -> Sum1/1
  Integrator1/1 -> Sum1/2, Out1/1
  Sum1/1 -> Gain/1
  Gain/1 -> Integrator1/1

== system test_sequence_lib/ac Network with MVT (native math)/solver_LPF1 ==
  In1 : Inport
  Gain : Gain  Gain=1/1e-3
  Integrator1 : Integrator
  Sum1 : Sum  Inputs=|+-
  Out1 : Outport
  wires:
  Gain/1 -> Integrator1/1
  Sum1/1 -> Gain/1
  Integrator1/1 -> Out1/1, Sum1/2
  In1/1 -> Sum1/1

== system test_sequence_lib/dcac SST cells/SST Cell Model ==
  v_LV : Inport
  i_MV : Inport  Port=2
  v_ac : Inport  Port=3
  i_ac : Inport  Port=4
  Gain1 : Gain  Gain=1/C_MV_CELL
  Integrator1 : Integrator
  Product : Product  Inputs=*/
  Product1 : Product
  Product2 : Product
  Product5 : Product  Inputs=*/
  Saturation1 : Saturate  UpperLimit=inf  LowerLimit=50
  Saturation3 : Saturate  UpperLimit=inf  LowerLimit=500
  Sum1 : Sum  Inputs=|+-
  v_MV_cell : Outport
  i_LV : Outport  Port=2
  wires:
  Integrator1/1 -> v_MV_cell/1, Saturation3/1, Product1/2  "v_MV_cell"
  Saturation3/1 -> Product5/2
  v_LV/1 -> Saturation1/1
  Gain1/1 -> Integrator1/1
  Product5/1 -> Sum1/2  "i_mv_dcac"
  Product1/1 -> Product/1
  Sum1/1 -> Gain1/1
  i_MV/1 -> Product1/1, Sum1/1
  Product2/1 -> Product5/1  "p_inv_cell"
  i_ac/1 -> Product2/2
  v_ac/1 -> Product2/1
  Product/1 -> i_LV/1
  Saturation1/1 -> Product/2

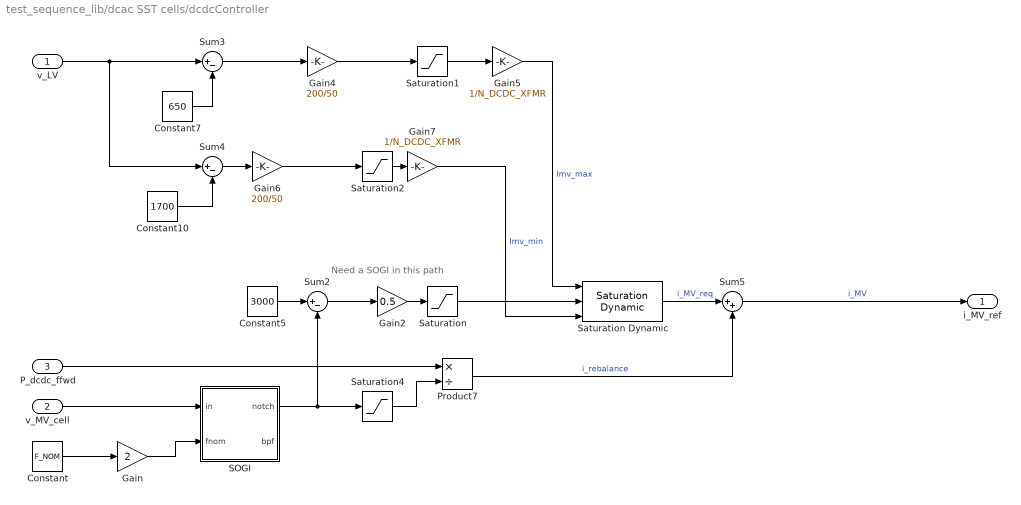
== system test_sequence_lib/dcac SST cells/dcdcController ==
  note: Need a SOGI in this path
  v_LV : Inport
  v_MV_cell : Inport  Port=2
  P_dcdc_ffwd : Inport  Port=3
  Constant : Constant  Value=F_NOM
  Constant10 : Constant  Value=1700
  Constant5 : Constant  Value=3000
  Constant7 : Constant  Value=650
  Gain : Gain  Gain=2
  Gain2 : Gain  Gain=0.5
  Gain4 : Gain  Gain=200/50
  Gain5 : Gain  Gain=1/N_DCDC_XFMR
  Gain6 : Gain  Gain=200/50
  Gain7 : Gain  Gain=1/N_DCDC_XFMR
  Product7 : Product  Inputs=*/
  SOGI : Subsystem
  Saturation : Saturate  UpperLimit=IMV_MAX  LowerLimit=IMV_MIN
  Saturation Dynamic : simulink/Discontinuities/Saturation Dynamic  OutMin=[]  OutMax=[]  OutDataTypeStr=Inherit: Same as second input  OutDataType=fixdt(1, 16)  OutScaling=2^-10  DoSatur=off
  Saturation1 : Saturate  UpperLimit=ILV_MAX  LowerLimit=ILV_MIN
  Saturation2 : Saturate  UpperLimit=ILV_MAX  LowerLimit=ILV_MIN
  Saturation4 : Saturate  UpperLimit=inf  LowerLimit=2000
  Sum2 : Sum  Inputs=|+-
  Sum3 : Sum  Inputs=|+-
  Sum4 : Sum  Inputs=|+-
  Sum5 : Sum  Inputs=|++
  i_MV_ref : Outport
  wires:
  Constant10/1 -> Sum4/2
  Sum2/1 -> Gain2/1
  SOGI/1(notch) -> Sum2/2, Saturation4/1
  Gain4/1 -> Saturation1/1
  Saturation/1 -> Saturation Dynamic/2
  Gain2/1 -> Saturation/1
  Constant7/1 -> Sum3/2
  v_LV/1 -> Sum3/1, Sum4/1
  Constant5/1 -> Sum2/1
  Saturation1/1 -> Gain5/1
  Saturation Dynamic/1 -> Sum5/1  "i_MV_req"
  Sum4/1 -> Gain6/1
  Gain6/1 -> Saturation2/1
  Product7/1 -> Sum5/2  "i_rebalance"
  Gain7/1 -> Saturation Dynamic/3  "Imv_min"
  P_dcdc_ffwd/1 -> Product7/1
  Gain5/1 -> Saturation Dynamic/1  "Imv_max"
  Saturation2/1 -> Gain7/1
  Sum3/1 -> Gain4/1
  Saturation4/1 -> Product7/2
  Sum5/1 -> i_MV_ref/1  "i_MV"
  Gain/1 -> SOGI/2(fnom)
  v_MV_cell/1 -> SOGI/1(in)
  Constant/1 -> Gain/1

== system test_sequence_lib/grid_voltage/oscillator_3ph ==
  f : Inport
  phase : Inport  Port=2
  Cos : Trigonometry  Operator=cos
  Gain : Gain  Gain=2*pi
  Integrator : Integrator
  Real-Imag to Complex : RealImagToComplex
  Sin : Trigonometry
  Sum1 : Sum  Inputs=|++
  Sum2 : Sum  Inputs=|++
  phase_shift : Constant  Value=[0 -1/3 -2/3]
  osc[3] : Outport
  wires:
  Sum1/1 -> Gain/1
  Sin/1 -> Real-Imag to Complex/2
  Integrator/1 -> Sum1/1
  Sum2/1 -> Sin/1, Cos/1
  Cos/1 -> Real-Imag to Complex/1
  Real-Imag to Complex/1 -> osc[3]/1
  f/1 -> Integrator/1
  phase_shift/1 -> Sum1/2
  phase/1 -> Sum2/2
  Gain/1 -> Sum2/1

== system test_sequence_lib/AcMeter/PLL_3ph/SOGI ==
  in : Inport
  fnom : Inport  Port=2
  2pi : Gain  Gain=2*pi
  Integrator2 : Integrator
  Integrator3 : Integrator
  Product : Product
  Product1 : Product
  Sum4 : Sum  Inputs=|+-
  Sum5 : Sum  Inputs=|+-
  alpha : Gain  Gain=0.1
  notch : Outport
  bpf : Outport  Port=2
  wires:
  Product1/1 -> Integrator3/1
  Product/1 -> Integrator2/1
  2pi/1 -> Product/2, Product1/2
  Integrator3/1 -> Sum4/2
  Sum4/1 -> Product/1
  Sum5/1 -> notch/1, alpha/1
  alpha/1 -> Sum4/1
  Integrator2/1 -> bpf/1, Sum5/2, Product1/1
  fnom/1 -> 2pi/1
  in/1 -> Sum5/1

== system test_sequence_lib/AcMeter/PLL_3ph/oscillator_3ph ==
  f : Inport
  Cos : Trigonometry  Operator=cos
  Gain : Gain  Gain=2*pi
  Integrator : Integrator
  Real-Imag to Complex : RealImagToComplex
  Sin : Trigonometry
  Sum1 : Sum  Inputs=|++
  phase_shift : Constant  Value=[0 -1/3 -2/3]
  osc[3] : Outport
  wires:
  Sum1/1 -> Gain/1
  phase_shift/1 -> Sum1/2
  Sin/1 -> Real-Imag to Complex/2
  Integrator/1 -> Sum1/1
  Gain/1 -> Sin/1, Cos/1
  Cos/1 -> Real-Imag to Complex/1
  Real-Imag to Complex/1 -> osc[3]/1
  f/1 -> Integrator/1

== system test_sequence_lib/AcMeter/phasor_analysis/complex_LPF1 ==
  In1 : Inport
  Complex to Real-Imag : ComplexToRealImag
  Integrator : Integrator
  Integrator1 : Integrator
  Real-Imag to Complex : RealImagToComplex
  Sum1 : Sum  Inputs=|+-
  Sum2 : Sum  Inputs=|+-
  wLPF : Gain  Gain=wLPF
  wLPF1 : Gain  Gain=wLPF
  1 : Outport
  wires:
  Complex to Real-Imag/1 -> Sum1/1
  Sum1/1 -> wLPF/1
  wLPF/1 -> Integrator/1
  Integrator/1 -> Sum1/2, Real-Imag to Complex/1
  In1/1 -> Complex to Real-Imag/1
  Real-Imag to Complex/1 -> 1/1
  Integrator1/1 -> Real-Imag to Complex/2, Sum2/2
  wLPF1/1 -> Integrator1/1
  Sum2/1 -> wLPF1/1
  Complex to Real-Imag/2 -> Sum2/1

== system test_sequence_lib/dcac SST cells/dcdcController/SOGI ==
  in : Inport
  fnom : Inport  Port=2
  2pi : Gain  Gain=2*pi
  Integrator2 : Integrator
  Integrator3 : Integrator
  Product : Product
  Product1 : Product
  Sum4 : Sum  Inputs=|+-
  Sum5 : Sum  Inputs=|+-
  alpha : Gain
  notch : Outport
  bpf : Outport  Port=2
  wires:
  Product1/1 -> Integrator3/1
  Product/1 -> Integrator2/1
  2pi/1 -> Product/2, Product1/2
  Integrator3/1 -> Sum4/2
  Sum4/1 -> Product/1
  Sum5/1 -> notch/1, alpha/1
  alpha/1 -> Sum4/1
  Integrator2/1 -> bpf/1, Sum5/2, Product1/1
  fnom/1 -> 2pi/1
  in/1 -> Sum5/1
